simulink model "afe_rst_inv_psm_distributed_control_two_delays"  (R2026a)
settings: Solver=ode1be  StopTime=simlength  FixedStep=tc  MaxStep=Tc
values from neighbouring files (symbols this model uses):
  Amplitude_U = 1.16    [grid_fault_generator.m]
  Amplitude_V = Amplitude_U    (= 1.16)    [grid_fault_generator.m]
  Amplitude_W = Amplitude_U    (= 1.16)    [grid_fault_generator.m]
  end_time_LVRT = start_time_LVRT + error_length    [grid_fault_generator.m]
  Igrid_phase_normalization_factor = 270*sqrt(2)    [grid_emulator.m]
  omega_grid_emulator_nom = w_grid    (= 314.159265359)    [grid_emulator.m]
  omega_grid_nom = w_grid    (= 314.159265359)    [grid_emulator.m]
  t_ramp = 20e-3    (= 0.02)    [grid_fault_generator.m]
  ugrid_factor = 1    [grid_emulator.m]
  V_phase_normalization_factor = Vgrid_phase_normalization_factor    [grid_emulator.m]
  Vdc_bez = 1070    [grid_emulator.m]
  Vemu_ref_norm = Vemu_ref * sqrt(2) / V_phase_normalization_factor    [grid_emulator.m]
  vn_eta_pu = 0    [grid_emulator.m]
  vn_xi_pu = 0    [grid_emulator.m]
  vp_xi_pu = 1    [grid_emulator.m]
undefined symbols (not defined in the file or in its folder): Adrso, Aresd, Bresd, CFi, CFu, Cresd, Crso, CTRPIFF_CLIP_RELEASE, dead_time_INV, emf_fb_p, emf_fb_p_ccaller_1, emf_fb_p_ccaller_2, emf_p, emf_p_ccaller_1, emf_p_ccaller_2, fPWM_INV, g0_161Hz, g0_500Hz, g1_161Hz, g1_500Hz, i_grid_neg_eta_lim, i_grid_neg_eta_red_lim, i_grid_neg_xi_lim, i_grid_neg_xi_red_lim, i_grid_pos_eta_lim, i_grid_pos_eta_red_lim, ibez, id_lim, ieta_neg_ref_lim, ieta_pos_ref_lim, iq_lim, ixi_pos_ref_lim, Jm_norm, k_frt_ref, kg, ki_afe, ki_i, ki_id, ki_iq, ki_rc_neg_grid, ki_rc_pos_grid, ki_vs, ki_w, kp_afe, kp_i, kp_id, kp_iq, kp_rc_neg_grid, kp_rc_pos_grid, kp_vs, kp_w, kw, l1, l2, Lalpha_norm, Ld_norm, Ldrso, Lq_norm, Ls_norm, luenberger_l1 ... (+30)
libraries: fl_lib x146, nesl_utility x62, simulink x8, cstblocks_lti x7, sl_discontinuities x3, single_phase_transformer_lib x3, flexshaft_lib x1, permanent_magnet_synchronous_machine x1
(part 13 of 14)

== system afe_rst_inv_psm_distributed_control_two_delays/INV-Modular/inv_leg_v/driver_board_v/motor_vector_control/bemf_observer/bemf_observer_simulink/double_integrator_observer ==
  theta : Inport
  Gain : Gain  Gain=kw
  Gain1 : Gain  Gain=kg
  Gain2 : Gain  Gain=omega_bez
  Gain3 : Gain  Gain=1/omega_bez
  Gain5 : Gain  Gain=ts_inv
  Sum : Sum  Inputs=-+|
  Sum1 : Sum  Inputs=|++
  Sum2 : Sum  Inputs=|++
  Sum8 : Sum  Inputs=++|
  Unit Delay1 : UnitDelay  SampleTime=ts_inv
  Unit Delay2 : UnitDelay  SampleTime=ts_inv
  bounder1 : MATLAB Function  TreatAsAtomicUnit=on  SystemSampleTime=ts_inv
  bounder2 : MATLAB Function  TreatAsAtomicUnit=on  SystemSampleTime=ts_inv
  omega_pu_hat : Outport  VectorParamsAs1DForOutWhenUnconnected=off
  theta_hat : Outport  Port=2  VectorParamsAs1DForOutWhenUnconnected=off
  tag scope: theta_hat_dbv=global
  wires:
  Unit Delay1/1 -> Sum/1, theta_hat/1, Sum2/2, [theta_hat_dbv]  "theta_hat"
  Sum/1 -> bounder1/1(u)
  Gain5/1 -> Gain2/1
  Gain3/1 -> Sum1/1
  Gain2/1 -> Sum8/1
  bounder1/1(y) -> Gain1/1, Gain/1
  bounder2/1(y) -> Unit Delay1/1
  Sum2/1 -> Sum8/2
  Unit Delay2/1 -> Gain5/1, Sum1/2, omega_pu_hat/1
  Gain/1 -> Gain3/1
  Sum1/1 -> Unit Delay2/1
  Sum8/1 -> bounder2/1(u)
  theta/1 -> Sum/2  "theta_bemf"
  Gain1/1 -> Sum2/1

== system afe_rst_inv_psm_distributed_control_two_delays/INV-Modular/inv_leg_v/driver_board_v/motor_vector_control/bemf_observer/bemf_observer_simulink/omega_hat_flt ==
  omega_hat : Inport
  Gain3 : Gain  Gain=omega_flt_g1
  Gain6 : Gain  Gain=omega_flt_g0
  Sum : Sum  Inputs=|++
  Unit Delay1 : UnitDelay  SampleTime=ts_inv
  omega_hat_flt : Outport  VectorParamsAs1DForOutWhenUnconnected=off
  wires:
  Sum/1 -> omega_hat_flt/1, Unit Delay1/1
  Gain3/1 -> Sum/2
  Unit Delay1/1 -> Gain3/1
  omega_hat/1 -> Gain6/1
  Gain6/1 -> Sum/1

== system afe_rst_inv_psm_distributed_control_two_delays/INV-Modular/inv_leg_v/driver_board_v/motor_vector_control/bemf_observer/bemf_observer_simulink/psi_alpha_hat ==
  ualpha : Inport
  ialpha : Inport  Port=2
  Gain1 : Gain  Gain=Rs_norm
  Gain2 : Gain  Gain=emf_fb_p
  Gain3 : Gain  Gain=emf_p
  Gain4 : Gain  Gain=omega_bez
  Gain5 : Gain  Gain=Ls_norm
  Gain6 : Gain  Gain=motorc_m_scale
  Gain7 : Gain  Gain=ts_inv
  Product : Product  RndMeth=Zero
  Sum : Sum  Inputs=|+-
  Sum1 : Sum  Inputs=|+-
  Sum2 : Sum  Inputs=++-  SaturateOnIntegerOverflow=on
  Sum3 : Sum  Inputs=|++
  Sum4 : Sum  Inputs=+-  SaturateOnIntegerOverflow=on
  Unit Delay1 : UnitDelay  SampleTime=ts_inv
  Unit Delay2 : UnitDelay  SampleTime=ts_inv
  psi_s_alpha_hat : Outport  VectorParamsAs1DForOutWhenUnconnected=off
  psi_r_alpha_hat : Outport  Port=2  VectorParamsAs1DForOutWhenUnconnected=off
  tag scope: psi_r_alpha_hat_dbv=global
  wires:
  Gain5/1 -> Sum4/2
  Gain6/1 -> Sum/1
  Product/1 -> Gain6/1
  Gain7/1 -> Sum3/1
  [udc_pu_dbv] -> Product/2
  Gain2/1 -> Sum2/1
  Sum1/1 -> Gain2/1
  Sum3/1 -> Unit Delay1/1  "psi_s_alpha_hat_hat"
  Unit Delay1/1 -> psi_s_alpha_hat/1, Sum4/1, Sum3/2, Gain3/1
  ualpha/1 -> Product/1
  Sum/1 -> Sum2/2
  Gain1/1 -> Sum/2
  ialpha/1 -> Gain1/1, Gain5/1
  Gain3/1 -> Sum2/3
  Sum2/1 -> Gain4/1
  Gain4/1 -> Gain7/1
  [psi_r_alpha_hat_dbv] -> Sum1/2
  [psi_r_m_alpha_dbv] -> Sum1/1
  Sum4/1 -> Unit Delay2/1
  Unit Delay2/1 -> [psi_r_alpha_hat_dbv], psi_r_alpha_hat/1

== system afe_rst_inv_psm_distributed_control_two_delays/INV-Modular/inv_leg_v/driver_board_v/motor_vector_control/bemf_observer/bemf_observer_simulink/psi_beta_hat ==
  ubeta : Inport
  ibeta : Inport  Port=2
  Gain1 : Gain  Gain=Rs_norm
  Gain2 : Gain  Gain=emf_fb_p
  Gain3 : Gain  Gain=emf_p
  Gain4 : Gain  Gain=omega_bez
  Gain5 : Gain  Gain=Ls_norm
  Gain6 : Gain  Gain=motorc_m_scale
  Gain7 : Gain  Gain=ts_inv
  Product : Product  RndMeth=Zero
  Sum : Sum  Inputs=|+-
  Sum1 : Sum  Inputs=|+-
  Sum2 : Sum  Inputs=++-  SaturateOnIntegerOverflow=on
  Sum3 : Sum  Inputs=|++
  Sum4 : Sum  Inputs=+-  SaturateOnIntegerOverflow=on
  Unit Delay1 : UnitDelay  SampleTime=ts_inv
  Unit Delay2 : UnitDelay  SampleTime=ts_inv
  psi_s_beta_hat : Outport  VectorParamsAs1DForOutWhenUnconnected=off
  psi_r_beta_hat : Outport  Port=2  VectorParamsAs1DForOutWhenUnconnected=off
  tag scope: psi_r_beta_hat_dbv=global
  wires:
  Gain5/1 -> Sum4/2
  Gain6/1 -> Sum/1
  Product/1 -> Gain6/1
  Gain7/1 -> Sum3/1
  [udc_pu_dbv] -> Product/2
  ubeta/1 -> Product/1
  Gain2/1 -> Sum2/1
  Sum3/1 -> Unit Delay1/1
  Unit Delay1/1 -> psi_s_beta_hat/1, Sum4/1, Sum3/2, Gain3/1
  [psi_r_m_beta_dbv] -> Sum1/1
  [psi_r_beta_hat_dbv] -> Sum1/2
  Sum1/1 -> Gain2/1
  Gain4/1 -> Gain7/1
  Sum2/1 -> Gain4/1
  Gain3/1 -> Sum2/3
  ibeta/1 -> Gain1/1, Gain5/1
  Gain1/1 -> Sum/2
  Sum/1 -> Sum2/2
  Sum4/1 -> Unit Delay2/1
  Unit Delay2/1 -> [psi_r_beta_hat_dbv], psi_r_beta_hat/1

== system afe_rst_inv_psm_distributed_control_two_delays/INV-Modular/inv_leg_v/driver_board_v/motor_vector_control/bemf_observer/bemf_observer_simulink/theta_bemf_hat ==
  psi_r_alpha_hat : Inport
  psi_r_beta_hat : Inport  Port=2
  omega_pu_hat : Inport  Port=3
  Sum : Sum  Inputs=|++
  Trigonometric Function : Trigonometry  Operator=atan2  OutputSignalType=real
  phase_compensation_omega : Gain  Gain=phase_compensation_omega
  theta_emf_hat : Outport  VectorParamsAs1DForOutWhenUnconnected=off
  wires:
  Sum/1 -> theta_emf_hat/1
  phase_compensation_omega/1 -> Sum/2
  omega_pu_hat/1 -> phase_compensation_omega/1
  Trigonometric Function/1 -> Sum/1
  psi_r_beta_hat/1 -> Trigonometric Function/1
  psi_r_alpha_hat/1 -> Trigonometric Function/2

== system afe_rst_inv_psm_distributed_control_two_delays/INV-Modular/inv_leg_v/driver_board_v/motor_vector_control/bemf_observer/bemf_observer_with_load_estimator_ccaller/Reset Trigger ==
  Step : Step  Time=0.01  InitialValue=1  FinalValue=0  SampleTime=0
  Out1 : Outport
  wires:
  Step/1 -> Out1/1  "Reset"

== system afe_rst_inv_psm_distributed_control_two_delays/INV-Modular/inv_leg_v/driver_board_v/motor_vector_control/current_ctrl/dq_pi_with_vector_antiwindup/dq_vector_pi ==
  id : Inport
  id_ref : Inport  Port=2
  iq : Inport  Port=3
  iq_ref : Inport  Port=4
  Sum1 : Sum  Inputs=|+-
  Sum2 : Sum  Inputs=|+-
  bounder1 : Subsystem
  bounder2 : Subsystem
  pi_d : Subsystem
  pi_q : Subsystem
  switch : Subsystem
  vector lenght : Subsystem
  ctrl_d_u : Outport
  ctrl_q_u : Outport  Port=2
  wires:
  bounder2/2(clip) -> switch/2(clip 2)
  bounder2/1(mq_sat) -> ctrl_q_u/1
  pi_q/1(Vqs_out) -> bounder2/3(mq), vector lenght/2(mq)
  vector lenght/1(m_1) -> bounder1/2(m_1), bounder2/2(m_1)
  vector lenght/2(m) -> bounder1/3(m), bounder2/1(m)
  pi_d/1(ud_out) -> vector lenght/1(md), bounder1/1(md)
  switch/1(clip) -> pi_q/2(clip), pi_d/2(clip)
  bounder1/2(clip) -> switch/1(clip 1)
  Sum2/1 -> pi_q/1(iq_tilde)
  Sum1/1 -> pi_d/1(id_tilde)
  bounder1/1(md_sat) -> ctrl_d_u/1
  id_ref/1 -> Sum1/1
  id/1 -> Sum1/2
  iq_ref/1 -> Sum2/1
  iq/1 -> Sum2/2

== system afe_rst_inv_psm_distributed_control_two_delays/INV-Modular/inv_leg_v/driver_board_v/motor_vector_control/current_ctrl/dq_pi_with_vector_antiwindup/dq_vector_pi_ccaller ==
  id : Inport
  id_ref : Inport  Port=2
  iq : Inport  Port=3
  iq_ref : Inport  Port=4
  Bus Selector : BusSelector  OutputSignals=ud,uq
  Constant : Constant  Value=ts_inv
  Constant1 : Constant  Value=kp_i
  Constant2 : Constant  Value=ki_i
  Constant3 : Constant  Value=pwm_out_lim
  Constant4 : Constant  Value=kp_i
  Constant5 : Constant  Value=ki_i
  Data Type Conversion{,1..2,4..6,9..13} (11 alike) : DataTypeConversion  OutDataTypeStr=single  SaturateOnIntegerOverflow=off  RndMeth=Floor
  Data Type Conversion3 : DataTypeConversion  OutDataTypeStr=double  SaturateOnIntegerOverflow=off  RndMeth=Floor
  Data Type Conversion7 : DataTypeConversion  OutDataTypeStr=double  SaturateOnIntegerOverflow=off  RndMeth=Floor
  Data Type Conversion8 : DataTypeConversion  OutDataTypeStr=uint8  SaturateOnIntegerOverflow=off  RndMeth=Floor
  Reset : Subsystem
  Zero-Order Hold{,1..11} (12 alike) : ZeroOrderHold  SampleTime=ts_inv
  dqpi_phase_v : CCaller  FunctionName=dqvector_pi_process_simulink  PortSpecificationStruct="%)30     .    ,!8   8    (     @         %    \"     T    !     0         %  0 \"0    $    _    07)G3F%M90  4&]R=$YA;64 4V-O<&4     26YD97@     5'EP90      4VEZ90      27-';&]B86P   X    P    !@    @    $          4    (     0    ,    !         !   P!O=70 #@   #     &    \"     0         !0    @    !     P    $         $  # &]U=  .    .     8    (    !          %    \"     $    &     0         0   ...(+7280 chars)"  SampleTime=ts_inv
  ud_ctrl_out : Outport
  uq_ctrl_out : Outport  Port=2
  wires:
  Data Type Conversion5/1 -> dqpi_phase_v/6
  Data Type Conversion/1 -> dqpi_phase_v/2
  dqpi_phase_v/1 -> Bus Selector/1  "out"
  Data Type Conversion1/1 -> dqpi_phase_v/3
  Data Type Conversion4/1 -> dqpi_phase_v/5
  Data Type Conversion2/1 -> dqpi_phase_v/4
  Data Type Conversion6/1 -> dqpi_phase_v/7
  Zero-Order Hold/1 -> Data Type Conversion6/1
  Zero-Order Hold5/1 -> Data Type Conversion/1
  Zero-Order Hold4/1 -> Data Type Conversion1/1
  Zero-Order Hold3/1 -> Data Type Conversion2/1
  Zero-Order Hold2/1 -> Data Type Conversion4/1
  Zero-Order Hold1/1 -> Data Type Conversion5/1
  [udc_pu_dba] -> Zero-Order Hold1/1
  Constant/1 -> Zero-Order Hold/1
  id_ref/1 -> Zero-Order Hold5/1
  iq_ref/1 -> Zero-Order Hold3/1
  id/1 -> Zero-Order Hold4/1
  iq/1 -> Zero-Order Hold2/1
  Bus Selector/2 -> Data Type Conversion3/1  "<uq>"
  Bus Selector/1 -> Data Type Conversion7/1  "<ud>"
  Data Type Conversion7/1 -> ud_ctrl_out/1  "ud"
  Data Type Conversion3/1 -> uq_ctrl_out/1  "uq"
  Reset/1(en) -> Zero-Order Hold11/1
  Data Type Conversion8/1 -> dqpi_phase_v/1
  Constant1/1 -> Zero-Order Hold6/1
  Zero-Order Hold6/1 -> Data Type Conversion9/1
  Data Type Conversion9/1 -> dqpi_phase_v/8
  Data Type Conversion10/1 -> dqpi_phase_v/9
  Zero-Order Hold7/1 -> Data Type Conversion10/1
  Zero-Order Hold8/1 -> Data Type Conversion11/1
  Constant2/1 -> Zero-Order Hold7/1
  Constant3/1 -> Zero-Order Hold8/1
  Data Type Conversion11/1 -> dqpi_phase_v/12
  Constant5/1 -> Zero-Order Hold10/1
  Zero-Order Hold10/1 -> Data Type Conversion12/1
  Zero-Order Hold9/1 -> Data Type Conversion13/1
  Constant4/1 -> Zero-Order Hold9/1
  Data Type Conversion13/1 -> dqpi_phase_v/10
  Data Type Conversion12/1 -> dqpi_phase_v/11
  Zero-Order Hold11/1 -> Data Type Conversion8/1

== system afe_rst_inv_psm_distributed_control_two_delays/INV-Modular/inv_leg_w/driver_board_w/motor_vector_control/bemf_observer/bemf_observer_ccaller/Reset Trigger ==
  Step : Step  Time=0.01  InitialValue=1  FinalValue=0  SampleTime=0
  Out1 : Outport
  wires:
  Step/1 -> Out1/1  "Reset"

== system afe_rst_inv_psm_distributed_control_two_delays/INV-Modular/inv_leg_w/driver_board_w/motor_vector_control/bemf_observer/bemf_observer_simulink/double_integrator_observer ==
  theta : Inport
  Gain : Gain  Gain=kw
  Gain1 : Gain  Gain=kg
  Gain2 : Gain  Gain=omega_bez
  Gain3 : Gain  Gain=1/omega_bez
  Gain5 : Gain  Gain=ts_inv
  Sum : Sum  Inputs=-+|
  Sum1 : Sum  Inputs=|++
  Sum2 : Sum  Inputs=|++
  Sum8 : Sum  Inputs=++|
  Unit Delay1 : UnitDelay  SampleTime=ts_inv
  Unit Delay2 : UnitDelay  SampleTime=ts_inv
  bounder1 : MATLAB Function  TreatAsAtomicUnit=on  SystemSampleTime=ts_inv
  bounder2 : MATLAB Function  TreatAsAtomicUnit=on  SystemSampleTime=ts_inv
  omega_pu_hat : Outport  VectorParamsAs1DForOutWhenUnconnected=off
  theta_hat : Outport  Port=2  VectorParamsAs1DForOutWhenUnconnected=off
  tag scope: theta_hat_dbw=global
  wires:
  Unit Delay1/1 -> Sum/1, theta_hat/1, Sum2/2, [theta_hat_dbw]  "theta_hat"
  Sum/1 -> bounder1/1(u)
  Gain5/1 -> Gain2/1
  Gain3/1 -> Sum1/1
  Gain2/1 -> Sum8/1
  bounder1/1(y) -> Gain1/1, Gain/1
  bounder2/1(y) -> Unit Delay1/1
  Sum2/1 -> Sum8/2
  Unit Delay2/1 -> Gain5/1, Sum1/2, omega_pu_hat/1
  Gain/1 -> Gain3/1
  Sum1/1 -> Unit Delay2/1
  Sum8/1 -> bounder2/1(u)
  theta/1 -> Sum/2  "theta_bemf"
  Gain1/1 -> Sum2/1

== system afe_rst_inv_psm_distributed_control_two_delays/INV-Modular/inv_leg_w/driver_board_w/motor_vector_control/bemf_observer/bemf_observer_simulink/omega_hat_flt ==
  omega_hat : Inport
  Gain3 : Gain  Gain=omega_flt_g1
  Gain6 : Gain  Gain=omega_flt_g0
  Sum : Sum  Inputs=|++
  Unit Delay1 : UnitDelay  SampleTime=ts_inv
  omega_hat_flt : Outport  VectorParamsAs1DForOutWhenUnconnected=off
  wires:
  Sum/1 -> omega_hat_flt/1, Unit Delay1/1
  Gain3/1 -> Sum/2
  Unit Delay1/1 -> Gain3/1
  omega_hat/1 -> Gain6/1
  Gain6/1 -> Sum/1

== system afe_rst_inv_psm_distributed_control_two_delays/INV-Modular/inv_leg_w/driver_board_w/motor_vector_control/bemf_observer/bemf_observer_simulink/psi_alpha_hat ==
  ualpha : Inport
  ialpha : Inport  Port=2
  Gain1 : Gain  Gain=Rs_norm
  Gain2 : Gain  Gain=emf_fb_p
  Gain3 : Gain  Gain=emf_p
  Gain4 : Gain  Gain=omega_bez
  Gain5 : Gain  Gain=Ls_norm
  Gain6 : Gain  Gain=motorc_m_scale
  Gain7 : Gain  Gain=ts_inv
  Product : Product  RndMeth=Zero
  Sum : Sum  Inputs=|+-
  Sum1 : Sum  Inputs=|+-
  Sum2 : Sum  Inputs=++-  SaturateOnIntegerOverflow=on
  Sum3 : Sum  Inputs=|++
  Sum4 : Sum  Inputs=+-  SaturateOnIntegerOverflow=on
  Unit Delay1 : UnitDelay  SampleTime=ts_inv
  Unit Delay2 : UnitDelay  SampleTime=ts_inv
  psi_s_alpha_hat : Outport  VectorParamsAs1DForOutWhenUnconnected=off
  psi_r_alpha_hat : Outport  Port=2  VectorParamsAs1DForOutWhenUnconnected=off
  tag scope: psi_r_alpha_hat_dbw=global
  wires:
  Gain5/1 -> Sum4/2
  Gain6/1 -> Sum/1
  Product/1 -> Gain6/1
  Gain7/1 -> Sum3/1
  [udc_pu_dbw] -> Product/2
  Gain2/1 -> Sum2/1
  Sum1/1 -> Gain2/1
  Sum3/1 -> Unit Delay1/1  "psi_s_alpha_hat_hat"
  Unit Delay1/1 -> psi_s_alpha_hat/1, Sum4/1, Sum3/2, Gain3/1
  ualpha/1 -> Product/1
  Sum/1 -> Sum2/2
  Gain1/1 -> Sum/2
  ialpha/1 -> Gain1/1, Gain5/1
  Gain3/1 -> Sum2/3
  Sum2/1 -> Gain4/1
  Gain4/1 -> Gain7/1
  [psi_r_alpha_hat_dbw] -> Sum1/2
  [psi_r_m_alpha_dbw] -> Sum1/1
  Sum4/1 -> Unit Delay2/1
  Unit Delay2/1 -> [psi_r_alpha_hat_dbw], psi_r_alpha_hat/1

== system afe_rst_inv_psm_distributed_control_two_delays/INV-Modular/inv_leg_w/driver_board_w/motor_vector_control/bemf_observer/bemf_observer_simulink/psi_beta_hat ==
  ubeta : Inport
  ibeta : Inport  Port=2
  Gain1 : Gain  Gain=Rs_norm
  Gain2 : Gain  Gain=emf_fb_p
  Gain3 : Gain  Gain=emf_p
  Gain4 : Gain  Gain=omega_bez
  Gain5 : Gain  Gain=Ls_norm
  Gain6 : Gain  Gain=motorc_m_scale
  Gain7 : Gain  Gain=ts_inv
  Product : Product  RndMeth=Zero
  Sum : Sum  Inputs=|+-
  Sum1 : Sum  Inputs=|+-
  Sum2 : Sum  Inputs=++-  SaturateOnIntegerOverflow=on
  Sum3 : Sum  Inputs=|++
  Sum4 : Sum  Inputs=+-  SaturateOnIntegerOverflow=on
  Unit Delay1 : UnitDelay  SampleTime=ts_inv
  Unit Delay2 : UnitDelay  SampleTime=ts_inv
  psi_s_beta_hat : Outport  VectorParamsAs1DForOutWhenUnconnected=off
  psi_r_beta_hat : Outport  Port=2  VectorParamsAs1DForOutWhenUnconnected=off
  tag scope: psi_r_beta_hat_dbw=global
  wires:
  Gain5/1 -> Sum4/2
  Gain6/1 -> Sum/1
  Product/1 -> Gain6/1
  Gain7/1 -> Sum3/1
  [udc_pu_dbw] -> Product/2
  ubeta/1 -> Product/1
  Gain2/1 -> Sum2/1
  Sum3/1 -> Unit Delay1/1
  Unit Delay1/1 -> psi_s_beta_hat/1, Sum4/1, Sum3/2, Gain3/1
  [psi_r_m_beta_dbw] -> Sum1/1
  [psi_r_beta_hat_dbw] -> Sum1/2
  Sum1/1 -> Gain2/1
  Gain4/1 -> Gain7/1
  Sum2/1 -> Gain4/1
  Gain3/1 -> Sum2/3
  ibeta/1 -> Gain1/1, Gain5/1
  Gain1/1 -> Sum/2
  Sum/1 -> Sum2/2
  Sum4/1 -> Unit Delay2/1
  Unit Delay2/1 -> [psi_r_beta_hat_dbw], psi_r_beta_hat/1

== system afe_rst_inv_psm_distributed_control_two_delays/INV-Modular/inv_leg_w/driver_board_w/motor_vector_control/bemf_observer/bemf_observer_simulink/theta_bemf_hat ==
  psi_r_alpha_hat : Inport
  psi_r_beta_hat : Inport  Port=2
  omega_pu_hat : Inport  Port=3
  Sum : Sum  Inputs=|++
  Trigonometric Function : Trigonometry  Operator=atan2  OutputSignalType=real
  phase_compensation_omega : Gain  Gain=phase_compensation_omega
  theta_emf_hat : Outport  VectorParamsAs1DForOutWhenUnconnected=off
  wires:
  Sum/1 -> theta_emf_hat/1
  phase_compensation_omega/1 -> Sum/2
  omega_pu_hat/1 -> phase_compensation_omega/1
  Trigonometric Function/1 -> Sum/1
  psi_r_beta_hat/1 -> Trigonometric Function/1
  psi_r_alpha_hat/1 -> Trigonometric Function/2

== system afe_rst_inv_psm_distributed_control_two_delays/INV-Modular/inv_leg_w/driver_board_w/motor_vector_control/bemf_observer/bemf_observer_with_load_estimator_ccaller/Reset Trigger ==
  Step : Step  Time=0.01  InitialValue=1  FinalValue=0  SampleTime=0
  Out1 : Outport
  wires:
  Step/1 -> Out1/1  "Reset"

== system afe_rst_inv_psm_distributed_control_two_delays/INV-Modular/inv_leg_w/driver_board_w/motor_vector_control/current_ctrl/dq_pi_with_vector_antiwindup/dq_vector_pi ==
  id : Inport
  id_ref : Inport  Port=2
  iq : Inport  Port=3
  iq_ref : Inport  Port=4
  Sum1 : Sum  Inputs=|+-
  Sum2 : Sum  Inputs=|+-
  bounder1 : Subsystem
  bounder2 : Subsystem
  pi_d : Subsystem
  pi_q : Subsystem
  switch : Subsystem
  vector lenght : Subsystem
  ctrl_d_u : Outport
  ctrl_q_u : Outport  Port=2
  wires:
  bounder2/2(clip) -> switch/2(clip 2)
  bounder2/1(mq_sat) -> ctrl_q_u/1
  pi_q/1(Vqs_out) -> bounder2/3(mq), vector lenght/2(mq)
  vector lenght/1(m_1) -> bounder1/2(m_1), bounder2/2(m_1)
  vector lenght/2(m) -> bounder1/3(m), bounder2/1(m)
  pi_d/1(ud_out) -> vector lenght/1(md), bounder1/1(md)
  switch/1(clip) -> pi_q/2(clip), pi_d/2(clip)
  bounder1/2(clip) -> switch/1(clip 1)
  Sum2/1 -> pi_q/1(iq_tilde)
  Sum1/1 -> pi_d/1(id_tilde)
  bounder1/1(md_sat) -> ctrl_d_u/1
  id_ref/1 -> Sum1/1
  id/1 -> Sum1/2
  iq_ref/1 -> Sum2/1
  iq/1 -> Sum2/2

== system afe_rst_inv_psm_distributed_control_two_delays/INV-Modular/inv_leg_w/driver_board_w/motor_vector_control/current_ctrl/dq_pi_with_vector_antiwindup/dq_vector_pi_ccaller ==
  id : Inport
  id_ref : Inport  Port=2
  iq : Inport  Port=3
  iq_ref : Inport  Port=4
  Bus Selector : BusSelector  OutputSignals=ud,uq
  Constant : Constant  Value=ts_inv
  Constant1 : Constant  Value=kp_id
  Constant2 : Constant  Value=ki_id
  Constant3 : Constant  Value=pwm_out_lim
  Constant4 : Constant  Value=kp_iq
  Constant5 : Constant  Value=ki_iq
  Data Type Conversion{,1..2,4..6,9..13} (11 alike) : DataTypeConversion  OutDataTypeStr=single  SaturateOnIntegerOverflow=off  RndMeth=Floor
  Data Type Conversion3 : DataTypeConversion  OutDataTypeStr=double  SaturateOnIntegerOverflow=off  RndMeth=Floor
  Data Type Conversion7 : DataTypeConversion  OutDataTypeStr=double  SaturateOnIntegerOverflow=off  RndMeth=Floor
  Data Type Conversion8 : DataTypeConversion  OutDataTypeStr=uint8  SaturateOnIntegerOverflow=off  RndMeth=Floor
  Reset : Subsystem
  Zero-Order Hold{,1..10} (11 alike) : ZeroOrderHold  SampleTime=ts_inv
  dqpi_phase_w : CCaller  FunctionName=dqvector_pi_process_simulink  PortSpecificationStruct="%)30     .    ,!8   8    (     @         %    \"     T    !     0         %  0 \"0    $    _    07)G3F%M90  4&]R=$YA;64 4V-O<&4     26YD97@     5'EP90      4VEZ90      27-';&]B86P   X    P    !@    @    $          4    (     0    ,    !         !   P!O=70 #@   #     &    \"     0         !0    @    !     P    $         $  # &]U=  .    .     8    (    !          %    \"     $    &     0         0   ...(+7280 chars)"  SampleTime=ts_inv
  ud_ctrl_out : Outport
  uq_ctrl_out : Outport  Port=2
  wires:
  Data Type Conversion5/1 -> dqpi_phase_w/6
  Data Type Conversion/1 -> dqpi_phase_w/2
  dqpi_phase_w/1 -> Bus Selector/1  "out"
  Data Type Conversion1/1 -> dqpi_phase_w/3
  Data Type Conversion4/1 -> dqpi_phase_w/5
  Data Type Conversion2/1 -> dqpi_phase_w/4
  Data Type Conversion6/1 -> dqpi_phase_w/7
  Zero-Order Hold/1 -> Data Type Conversion6/1
  Zero-Order Hold5/1 -> Data Type Conversion/1
  Zero-Order Hold4/1 -> Data Type Conversion1/1
  Zero-Order Hold3/1 -> Data Type Conversion2/1
  Zero-Order Hold2/1 -> Data Type Conversion4/1
  Zero-Order Hold1/1 -> Data Type Conversion5/1
  [udc_pu_dba] -> Zero-Order Hold1/1
  Constant/1 -> Zero-Order Hold/1
  id_ref/1 -> Zero-Order Hold5/1
  iq_ref/1 -> Zero-Order Hold3/1
  id/1 -> Zero-Order Hold4/1
  iq/1 -> Zero-Order Hold2/1
  Bus Selector/2 -> Data Type Conversion3/1  "<uq>"
  Bus Selector/1 -> Data Type Conversion7/1  "<ud>"
  Data Type Conversion7/1 -> ud_ctrl_out/1  "ud"
  Data Type Conversion3/1 -> uq_ctrl_out/1  "uq"
  Data Type Conversion8/1 -> dqpi_phase_w/1
  Constant1/1 -> Zero-Order Hold6/1
  Zero-Order Hold6/1 -> Data Type Conversion9/1
  Data Type Conversion9/1 -> dqpi_phase_w/8
  Data Type Conversion10/1 -> dqpi_phase_w/9
  Zero-Order Hold7/1 -> Data Type Conversion10/1
  Zero-Order Hold8/1 -> Data Type Conversion11/1
  Constant2/1 -> Zero-Order Hold7/1
  Constant3/1 -> Zero-Order Hold8/1
  Data Type Conversion11/1 -> dqpi_phase_w/12
  Constant5/1 -> Zero-Order Hold10/1
  Zero-Order Hold10/1 -> Data Type Conversion12/1
  Zero-Order Hold9/1 -> Data Type Conversion13/1
  Constant4/1 -> Zero-Order Hold9/1
  Data Type Conversion13/1 -> dqpi_phase_w/10
  Data Type Conversion12/1 -> dqpi_phase_w/11
  Reset/1(en) -> Data Type Conversion8/1

== system afe_rst_inv_psm_distributed_control_two_delays/INV-Modular/inv_leg_u/driver_board_u/motor_vector_control/current_ctrl/dq_pi_with_vector_antiwindup/dq_vector_pi/bounder1 ==
  md : Inport
  m_1 : Inport  Port=2
  m : Inport  Port=3
  Constant : Constant
  Constant1 : Constant  Value=0
  Divide : Product
  Switch : Switch  Threshold=pwm_out_lim  SaturateOnIntegerOverflow=off  InputSameDT=off
  Switch1 : Switch  Threshold=pwm_out_lim  SaturateOnIntegerOverflow=off  InputSameDT=off
  md_sat : Outport  VectorParamsAs1DForOutWhenUnconnected=off
  clip : Outport  Port=2  VectorParamsAs1DForOutWhenUnconnected=off
  wires:
  md/1 -> Switch1/3, Divide/2
  m_1/1 -> Divide/1
  Divide/1 -> Switch1/1
  Switch1/1 -> md_sat/1
  Switch/1 -> clip/1
  m/1 -> Switch/2, Switch1/2
  Constant/1 -> Switch/1
  Constant1/1 -> Switch/3

== system afe_rst_inv_psm_distributed_control_two_delays/INV-Modular/inv_leg_u/driver_board_u/motor_vector_control/current_ctrl/dq_pi_with_vector_antiwindup/dq_vector_pi/bounder2 ==
  m : Inport
  m_1 : Inport  Port=2
  mq : Inport  Port=3
  Constant : Constant
  Constant1 : Constant  Value=0
  Divide : Product
  Switch : Switch  Threshold=pwm_out_lim  SaturateOnIntegerOverflow=off  InputSameDT=off
  Switch1 : Switch  Threshold=pwm_out_lim  SaturateOnIntegerOverflow=off  InputSameDT=off
  mq_sat : Outport  VectorParamsAs1DForOutWhenUnconnected=off
  clip : Outport  Port=2  VectorParamsAs1DForOutWhenUnconnected=off
  wires:
  Constant1/1 -> Switch/3
  Constant/1 -> Switch/1
  m/1 -> Switch1/2, Switch/2
  Switch/1 -> clip/1
  Switch1/1 -> mq_sat/1
  Divide/1 -> Switch1/1
  m_1/1 -> Divide/1
  mq/1 -> Divide/2, Switch1/3

== system afe_rst_inv_psm_distributed_control_two_delays/INV-Modular/inv_leg_u/driver_board_u/motor_vector_control/current_ctrl/dq_pi_with_vector_antiwindup/dq_vector_pi/pi_d ==
  id_tilde : Inport
  clip : Inport  Port=2
  1/Ti : Gain  Gain=kp_id  SaturateOnIntegerOverflow=on  OutDataTypeStr=Inherit: Same as input  ParamDataTypeStr=Inherit: Same as input
  Constant : Constant  Value=0
  Constant1 : Constant  Value=Ls_norm
  Product : Product  Inputs=3
  Sum2 : Sum  Inputs=+-  SaturateOnIntegerOverflow=on
  Sum4 : Sum  SaturateOnIntegerOverflow=on
  Sum5 : Sum  Inputs=+++  SaturateOnIntegerOverflow=on
  Switch1 : Switch  Threshold=0.5  SaturateOnIntegerOverflow=off  InputSameDT=off
  Switch2 : Switch  Threshold=0.5  SaturateOnIntegerOverflow=off  InputSameDT=off
  Unit Delay1 : UnitDelay  SampleTime=ts_inv
  Unit Delay2 : UnitDelay  SampleTime=ts_inv
  kp1 : Gain  Gain=CTRPIFF_CLIP_RELEASE*ts_inv  SaturateOnIntegerOverflow=on  OutDataTypeStr=Inherit: Same as input  ParamDataTypeStr=Inherit: Same as input
  kp2 : Gain  Gain=ki_id*ts_inv  SaturateOnIntegerOverflow=on  OutDataTypeStr=Inherit: Same as input  ParamDataTypeStr=Inherit: Same as input
  kp3 : Gain  Gain=0  SaturateOnIntegerOverflow=on  OutDataTypeStr=Inherit: Same as input  ParamDataTypeStr=Inherit: Same as input
  ud_out : Outport  VectorParamsAs1DForOutWhenUnconnected=off
  wires:
  id_tilde/1 -> kp2/1, 1/Ti/1
  Switch1/1 -> Unit Delay2/1
  Sum4/1 -> Sum5/2, Switch1/3
  kp1/1 -> Sum2/2
  Sum2/1 -> Switch1/1
  Unit Delay2/1 -> Sum4/2, kp1/1, Sum2/1
  1/Ti/1 -> Sum5/1
  Switch2/1 -> Sum4/1
  kp2/1 -> Switch2/3
  clip/1 -> Unit Delay1/1
  [clip] -> Switch2/2
  [clip] -> Switch1/2
  Constant/1 -> Switch2/1
  Unit Delay1/1 -> [clip]
  Sum5/1 -> ud_out/1
  [iq_inverter_pu] -> Product/2
  [omega_pu_hat_flt] -> Product/1
  kp3/1 -> Sum5/3
  Constant1/1 -> Product/3
  Product/1 -> kp3/1

== system afe_rst_inv_psm_distributed_control_two_delays/INV-Modular/inv_leg_u/driver_board_u/motor_vector_control/current_ctrl/dq_pi_with_vector_antiwindup/dq_vector_pi/pi_q ==
  iq_tilde : Inport
  clip : Inport  Port=2
  1/Ti : Gain  Gain=kp_iq  SaturateOnIntegerOverflow=on  OutDataTypeStr=Inherit: Same as input  ParamDataTypeStr=Inherit: Same as input
  Constant : Constant  Value=0
  Constant1 : Constant  Value=Ls_norm
  Product : Product  Inputs=3
  Sum2 : Sum  Inputs=+-  SaturateOnIntegerOverflow=on
  Sum4 : Sum  SaturateOnIntegerOverflow=on
  Sum5 : Sum  Inputs=+++  SaturateOnIntegerOverflow=on
  Switch1 : Switch  Threshold=0.5  SaturateOnIntegerOverflow=off  InputSameDT=off
  Switch2 : Switch  Threshold=0.5  SaturateOnIntegerOverflow=off  InputSameDT=off
  Unit Delay1 : UnitDelay  SampleTime=ts_inv
  Unit Delay2 : UnitDelay  SampleTime=ts_inv
  kp1 : Gain  Gain=CTRPIFF_CLIP_RELEASE*ts_inv  SaturateOnIntegerOverflow=on  OutDataTypeStr=Inherit: Same as input  ParamDataTypeStr=Inherit: Same as input
  kp2 : Gain  Gain=ki_iq*ts_inv  SaturateOnIntegerOverflow=on  OutDataTypeStr=Inherit: Same as input  ParamDataTypeStr=Inherit: Same as input
  kp3 : Gain  Gain=0  SaturateOnIntegerOverflow=on  OutDataTypeStr=Inherit: Same as input  ParamDataTypeStr=Inherit: Same as input
  Vqs_out : Outport  VectorParamsAs1DForOutWhenUnconnected=off
  wires:
  Constant/1 -> Switch2/1
  [clip] -> Switch1/2
  [clip] -> Switch2/2
  clip/1 -> Unit Delay1/1
  kp2/1 -> Switch2/3
  Switch2/1 -> Sum4/1
  1/Ti/1 -> Sum5/1
  Unit Delay2/1 -> Sum2/1, kp1/1, Sum4/2
  Sum2/1 -> Switch1/1
  kp1/1 -> Sum2/2
  Sum4/1 -> Sum5/2, Switch1/3
  Switch1/1 -> Unit Delay2/1
  iq_tilde/1 -> 1/Ti/1, kp2/1
  Unit Delay1/1 -> [clip]
  Sum5/1 -> Vqs_out/1
  [omega_pu_hat_flt] -> Product/1
  [id_inverter_pu] -> Product/2
  Constant1/1 -> Product/3
  Product/1 -> kp3/1
  kp3/1 -> Sum5/3

== system afe_rst_inv_psm_distributed_control_two_delays/INV-Modular/inv_leg_u/driver_board_u/motor_vector_control/current_ctrl/dq_pi_with_vector_antiwindup/dq_vector_pi/switch ==
  clip 1 : Inport
  clip 2 : Inport  Port=2
  Constant4 : Constant
  Constant5 : Constant  Value=0
  Sum1 : Sum  SaturateOnIntegerOverflow=on
  Switch : Switch  Threshold=0.5  SaturateOnIntegerOverflow=off  InputSameDT=off
  clip : Outport  VectorParamsAs1DForOutWhenUnconnected=off
  wires:
  Constant5/1 -> Switch/3
  Switch/1 -> clip/1
  Constant4/1 -> Switch/1
  Sum1/1 -> Switch/2
  clip 1/1 -> Sum1/1
  clip 2/1 -> Sum1/2

== system afe_rst_inv_psm_distributed_control_two_delays/INV-Modular/inv_leg_u/driver_board_u/motor_vector_control/current_ctrl/dq_pi_with_vector_antiwindup/dq_vector_pi/vector lenght ==
  md : Inport
  mq : Inport  Port=2
  Math Function : Math  Operator=magnitude^2  SignedPower=on
  Math Function1 : Math  Operator=magnitude^2  SignedPower=on
  Math Function2 : Math  Operator=reciprocal  SignedPower=on
  Sqrt : Sqrt
  Sum5 : Sum  SaturateOnIntegerOverflow=on
  m_1 : Outport  VectorParamsAs1DForOutWhenUnconnected=off
  m : Outport  Port=2  VectorParamsAs1DForOutWhenUnconnected=off
  wires:
  Sqrt/1 -> m/1, Math Function2/1
  mq/1 -> Math Function1/1
  Math Function1/1 -> Sum5/2
  Math Function/1 -> Sum5/1
  Sum5/1 -> Sqrt/1
  Math Function2/1 -> m_1/1
  md/1 -> Math Function/1

== system afe_rst_inv_psm_distributed_control_two_delays/INV-Modular/inv_leg_u/driver_board_u/motor_vector_control/current_ctrl/dq_pi_with_vector_antiwindup/dq_vector_pi_ccaller/Reset ==
  Step : Step  Time=0.015  InitialValue=1  FinalValue=0  SampleTime=0
  en : Outport
  wires:
  Step/1 -> en/1

== system afe_rst_inv_psm_distributed_control_two_delays/INV-Modular/inv_leg_v/driver_board_v/motor_vector_control/current_ctrl/dq_pi_with_vector_antiwindup/dq_vector_pi/bounder1 ==
  md : Inport
  m_1 : Inport  Port=2
  m : Inport  Port=3
  Constant : Constant
  Constant1 : Constant  Value=0
  Divide : Product
  Switch : Switch  Threshold=pwm_out_lim  SaturateOnIntegerOverflow=off  InputSameDT=off
  Switch1 : Switch  Threshold=pwm_out_lim  SaturateOnIntegerOverflow=off  InputSameDT=off
  md_sat : Outport  VectorParamsAs1DForOutWhenUnconnected=off
  clip : Outport  Port=2  VectorParamsAs1DForOutWhenUnconnected=off
  wires:
  md/1 -> Switch1/3, Divide/2
  m_1/1 -> Divide/1
  Divide/1 -> Switch1/1
  Switch1/1 -> md_sat/1
  Switch/1 -> clip/1
  m/1 -> Switch/2, Switch1/2
  Constant/1 -> Switch/1
  Constant1/1 -> Switch/3

== system afe_rst_inv_psm_distributed_control_two_delays/INV-Modular/inv_leg_v/driver_board_v/motor_vector_control/current_ctrl/dq_pi_with_vector_antiwindup/dq_vector_pi/bounder2 ==
  m : Inport
  m_1 : Inport  Port=2
  mq : Inport  Port=3
  Constant : Constant
  Constant1 : Constant  Value=0
  Divide : Product
  Switch : Switch  Threshold=pwm_out_lim  SaturateOnIntegerOverflow=off  InputSameDT=off
  Switch1 : Switch  Threshold=pwm_out_lim  SaturateOnIntegerOverflow=off  InputSameDT=off
  mq_sat : Outport  VectorParamsAs1DForOutWhenUnconnected=off
  clip : Outport  Port=2  VectorParamsAs1DForOutWhenUnconnected=off
  wires:
  Constant1/1 -> Switch/3
  Constant/1 -> Switch/1
  m/1 -> Switch1/2, Switch/2
  Switch/1 -> clip/1
  Switch1/1 -> mq_sat/1
  Divide/1 -> Switch1/1
  m_1/1 -> Divide/1
  mq/1 -> Divide/2, Switch1/3

== system afe_rst_inv_psm_distributed_control_two_delays/INV-Modular/inv_leg_v/driver_board_v/motor_vector_control/current_ctrl/dq_pi_with_vector_antiwindup/dq_vector_pi/pi_d ==
  id_tilde : Inport
  clip : Inport  Port=2
  1/Ti : Gain  Gain=kp_id  SaturateOnIntegerOverflow=on  OutDataTypeStr=Inherit: Same as input  ParamDataTypeStr=Inherit: Same as input
  Constant : Constant  Value=0
  Constant1 : Constant  Value=Ls_norm
  Product : Product  Inputs=3
  Sum2 : Sum  Inputs=+-  SaturateOnIntegerOverflow=on
  Sum4 : Sum  SaturateOnIntegerOverflow=on
  Sum5 : Sum  Inputs=+++  SaturateOnIntegerOverflow=on
  Switch1 : Switch  Threshold=0.5  SaturateOnIntegerOverflow=off  InputSameDT=off
  Switch2 : Switch  Threshold=0.5  SaturateOnIntegerOverflow=off  InputSameDT=off
  Unit Delay1 : UnitDelay  SampleTime=ts_inv
  Unit Delay2 : UnitDelay  SampleTime=ts_inv
  kp1 : Gain  Gain=CTRPIFF_CLIP_RELEASE*ts_inv  SaturateOnIntegerOverflow=on  OutDataTypeStr=Inherit: Same as input  ParamDataTypeStr=Inherit: Same as input
  kp2 : Gain  Gain=ki_id*ts_inv  SaturateOnIntegerOverflow=on  OutDataTypeStr=Inherit: Same as input  ParamDataTypeStr=Inherit: Same as input
  kp3 : Gain  Gain=0  SaturateOnIntegerOverflow=on  OutDataTypeStr=Inherit: Same as input  ParamDataTypeStr=Inherit: Same as input
  ud_out : Outport  VectorParamsAs1DForOutWhenUnconnected=off
  wires:
  id_tilde/1 -> kp2/1, 1/Ti/1
  Switch1/1 -> Unit Delay2/1
  Sum4/1 -> Sum5/2, Switch1/3
  kp1/1 -> Sum2/2
  Sum2/1 -> Switch1/1
  Unit Delay2/1 -> Sum4/2, kp1/1, Sum2/1
  1/Ti/1 -> Sum5/1
  Switch2/1 -> Sum4/1
  kp2/1 -> Switch2/3
  clip/1 -> Unit Delay1/1
  [clip] -> Switch2/2
  [clip] -> Switch1/2
  Constant/1 -> Switch2/1
  Unit Delay1/1 -> [clip]
  Sum5/1 -> ud_out/1
  [iq_inverter_pu] -> Product/2
  [omega_pu_hat_flt] -> Product/1
  kp3/1 -> Sum5/3
  Constant1/1 -> Product/3
  Product/1 -> kp3/1
